simulink library "sm_robot_run_4legs_lib"  (R2025a)
settings: Solver=ode45  StartTime=0.0  StopTime=10.0  RelTol=1e-3
values from neighbouring files (symbols this model uses):
  N = 100    [Extr_Data_Cam_Roller_Curve.m]
  s = sin(q)    [Extr_Data_Cam_Roller_Curve.m]
undefined symbols (not defined in the file or in its folder): bw, d2r, Extr_Data_LinkEndHole, ground, J, joint_damping, k2, knee_torque, l1, l2, L_back, m1, m2, r2d, T_cg, t_th, t_w, th2, Trq_propulsive, u_th, u_w, X, Y, Z
libraries: sm_lib x25, nesl_utility x14, fl_lib x13, Contact_Forces_Lib x1, ee_lib x1
(part 2 of 2)

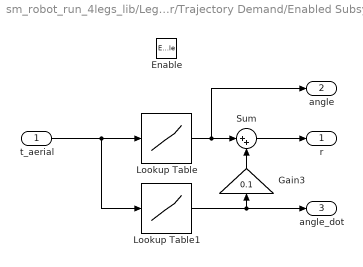
== system sm_robot_run_4legs_lib/Leg/Hip Actuator/Trajectory Demand/Enabled Subsystem ==
  t_aerial : Inport
  Enable : EnablePort  StatesWhenEnabling=reset
  Gain3 : Gain  Gain=0.1
  Lookup Table : Lookup  InputValues=t_th  Table=u_th  LookUpMeth=Interpolation-Use End Values  SaturateOnIntegerOverflow=off
  Lookup Table1 : Lookup  InputValues=t_w  Table=u_w  LookUpMeth=Interpolation-Use End Values  SaturateOnIntegerOverflow=off
  Sum : Sum  Inputs=|++
  r : Outport  OutputWhenDisabled=reset  InitialOutput=[0]  VectorParamsAs1DForOutWhenUnconnected=off
  angle : Outport  Port=2  OutputWhenDisabled=reset  InitialOutput=[0]  VectorParamsAs1DForOutWhenUnconnected=off
  angle_dot : Outport  Port=3  OutputWhenDisabled=reset  InitialOutput=[0]  VectorParamsAs1DForOutWhenUnconnected=off
  wires:
  Lookup Table1/1 -> angle_dot/1, Gain3/1
  t_aerial/1 -> Lookup Table/1, Lookup Table1/1
  Lookup Table/1 -> angle/1, Sum/1
  Sum/1 -> r/1
  Gain3/1 -> Sum/2

== system sm_robot_run_4legs_lib/Leg/Knee Actuator/Torque for knee retraction/Enabled Subsystem ==
  t_aerial : Inport
  Enable : EnablePort  StatesWhenEnabling=reset
  Angle profile : Subsystem
  Terminator1 : Terminator
  Torque Lookup Table : Lookup  InputValues=knee_torque.time  Table=knee_torque.signals.values  LookUpMeth=Interpolation-Use End Values  SaturateOnIntegerOverflow=off
  angle : Outport  OutputWhenDisabled=reset  InitialOutput=[0]  VectorParamsAs1DForOutWhenUnconnected=off
  wires:
  Angle profile/1(y) -> angle/1
  t_aerial/1 -> Angle profile/1(time), Torque Lookup Table/1
  Torque Lookup Table/1 -> Terminator1/1

== system sm_robot_run_4legs_lib/Leg/Contact Force Model/Planar/Force Law/Capture floor x-position ==
  x : Inport
  Trigger : TriggerPort  VariantControl=Variant
  x0 : Outport  InitialOutput=x0  VectorParamsAs1DForOutWhenUnconnected=off
  wires:
  x/1 -> x0/1

== system sm_robot_run_4legs_lib/Leg/Contact Force Model/Planar/Force Law/Penalty Force ==
  pen : Inport
  vel : Inport  Port=2
  Action Port : ActionPort
  Gain : Gain  Gain=[-ground.stiffness 0 0;0 -ground.stiffness 0;0 0 0]  Multiplication=Matrix(K*u)  SaturateOnIntegerOverflow=on  OutDataTypeStr=Inherit: Same as input  ParamDataTypeStr=Inherit: Same as input
  Gain1 : Gain  Gain=[-ground.damping 0 0;0 -ground.damping 0;0 0 0]  Multiplication=Matrix(K*u)  SaturateOnIntegerOverflow=on  OutDataTypeStr=Inherit: Same as input  ParamDataTypeStr=Inherit: Same as input
  Saturation : Saturate  UpperLimit=[inf inf inf]  LowerLimit=[-inf 0 -inf]
  Sum : Sum  Inputs=|++  SaturateOnIntegerOverflow=on
  force : Outport  InitialOutput=0  VectorParamsAs1DForOutWhenUnconnected=off
  wires:
  pen/1 -> Gain/1
  Gain/1 -> Sum/1
  Sum/1 -> Saturation/1
  Gain1/1 -> Sum/2
  vel/1 -> Gain1/1
  Saturation/1 -> force/1

== system sm_robot_run_4legs_lib/Leg/Contact Force Model/Planar/Force Law/Zero Force ==
  Action Port : ActionPort
  Zero Force : Constant  Value=[0;0;0]
  force : Outport  InitialOutput=0  VectorParamsAs1DForOutWhenUnconnected=off
  wires:
  Zero Force/1 -> force/1

== system sm_robot_run_4legs_lib/Leg/Knee Actuator/Torque for knee retraction/Enabled Subsystem/Angle profile ==
  time : Inport
  Constant angle t >= 6*T_cg/4 : Constant  Value=0
  Gain : Gain  Gain=-1
  Half sine wave 0 < t < 6*T_cg/4 : Subsystem
  Switch : Switch  Threshold=6*T_cg/4  SaturateOnIntegerOverflow=off  InputSameDT=off
      settings: AttributesFormatString=Threshold = %<Threshold>
  y : Outport  VectorParamsAs1DForOutWhenUnconnected=off
  wires:
  Gain/1 -> y/1
  time/1 -> Half sine wave 0 < t < 6*T_cg/4/1(time), Switch/2
  Half sine wave 0 < t < 6*T_cg/4/1(y) -> Switch/3
  Constant angle t >= 6*T_cg/4/1 -> Switch/1
  Switch/1 -> Gain/1

== system sm_robot_run_4legs_lib/Leg/Knee Actuator/Torque for knee retraction/Enabled Subsystem/Angle profile/Half sine wave 0 < t < 6*T_cg//4 ==
  time : Inport
  A : Gain  Gain=50
  Constant2 : Constant  Value=th2*r2d*0
  Sum : Sum  Inputs=++|
  sin(wt) : Trigonometry
  w : Gain  Gain=2*pi/(3*T_cg)
  y : Outport  VectorParamsAs1DForOutWhenUnconnected=off
  wires:
  time/1 -> w/1
  Sum/1 -> y/1
  Constant2/1 -> Sum/1
  A/1 -> Sum/2
  sin(wt)/1 -> A/1
  w/1 -> sin(wt)/1
